simulink model "control_clasic"  (R2025b)
settings: Solver=VariableStepAuto  StartTime=0.0  StopTime=10  RelTol=1e-3
libraries: slpidlib x2
settings Model: Creator=bogdu  LastModifiedBy=Sficaro

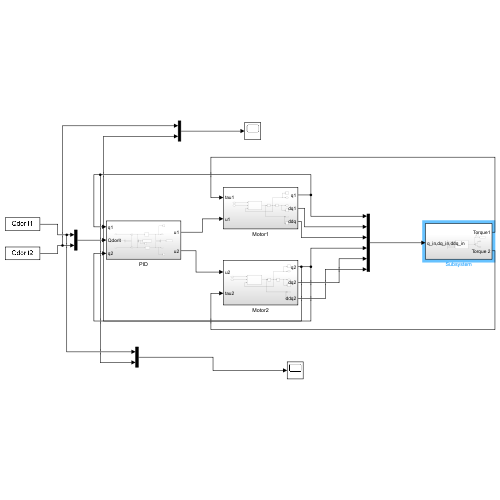
[thumbnail: Simulink's stored preview of the top-level diagram]
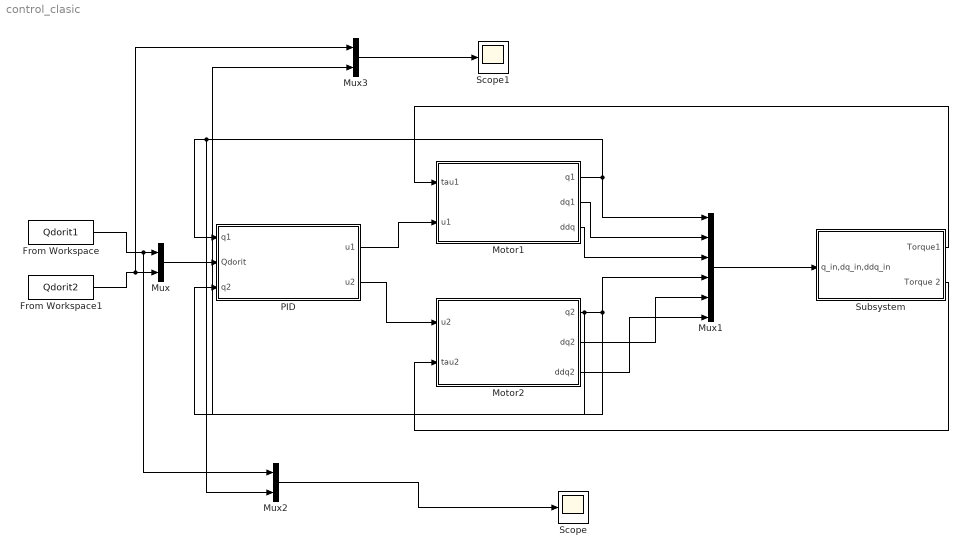
== system control_clasic ==
  From Workspace : FromWorkspace  VariableName=Qdorit1
  From Workspace1 : FromWorkspace  VariableName=Qdorit2
  Motor1 : Subsystem
  Motor2 : Subsystem
  Mux : Mux  Inputs=2
  Mux1 : Mux  Inputs=6
  Mux2 : Mux  Inputs=2
  Mux3 : Mux  Inputs=2
  PID : Subsystem
  Scope : Scope
      settings: ActiveDisplayYMinimum=-1  ActiveDisplayYMaximum=1  DataLoggingVariableName=ScopeData8
  Scope1 : Scope
      settings: ActiveDisplayYMinimum=-0.012500000000000004  ActiveDisplayYMaximum=0.11250000000000007
  Subsystem : Subsystem
  wires:
  From Workspace/1 -> Mux2/1, Mux/1
  From Workspace1/1 -> Mux3/1, Mux/2
  Mux/1 -> PID/2(Qdorit)
  Subsystem/1(Torque1) -> Motor1/1(tau1)
  Subsystem/2(Torque 2) -> Motor2/2(tau2)
  PID/1(u1) -> Motor1/2(u1)
  PID/2(u2) -> Motor2/1(u2)
  Motor1/1(q1) -> Mux1/1, Mux2/2, PID/1(q1)
  Motor2/1(q2) -> Mux3/2, Mux1/4, PID/3(q2)
  Motor1/2(dq1) -> Mux1/2
  Motor1/3(ddq) -> Mux1/3
  Motor2/2(dq2) -> Mux1/5
  Motor2/3(ddq2) -> Mux1/6
  Mux1/1 -> Subsystem/1(q_in,dq_in,ddq_in)
  Mux2/1 -> Scope/1
  Mux3/1 -> Scope1/1

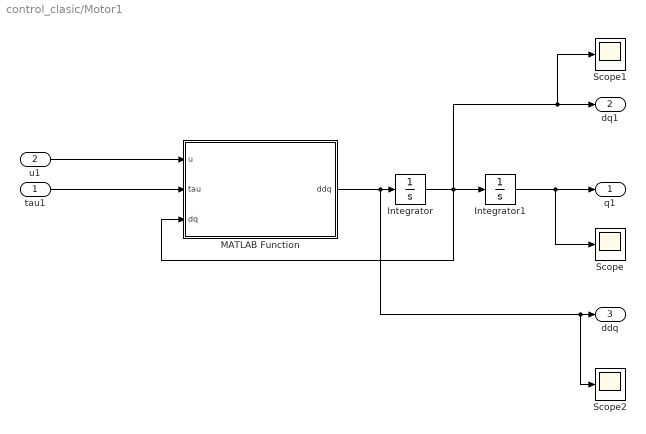
== system control_clasic/Motor1 ==
  tau1 : Inport
  u1 : Inport  Port=2
  Integrator : Integrator
  Integrator1 : Integrator
  MATLAB Function : MATLAB Function  TreatAsAtomicUnit=on
  Scope : Scope
      settings: ActiveDisplayYMinimum=-1  ActiveDisplayYMaximum=1
  Scope1 : Scope
      settings: ActiveDisplayYMinimum=-1  ActiveDisplayYMaximum=1
  Scope2 : Scope
      settings: ActiveDisplayYMinimum=-1  ActiveDisplayYMaximum=1  DataLoggingVariableName=ScopeData2
  q1 : Outport
  dq1 : Outport  Port=2
  ddq : Outport  Port=3
  wires:
  MATLAB Function/1(ddq) -> Scope2/1, ddq/1, Integrator/1
  Integrator1/1 -> Scope/1, q1/1
  Integrator/1 -> Scope1/1, dq1/1, Integrator1/1, MATLAB Function/3(dq)
  u1/1 -> MATLAB Function/1(u)
  tau1/1 -> MATLAB Function/2(tau)

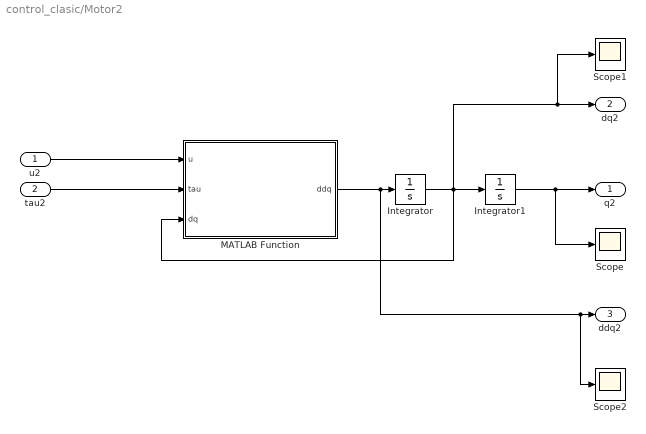
== system control_clasic/Motor2 ==
  u2 : Inport
  tau2 : Inport  Port=2
  Integrator : Integrator
  Integrator1 : Integrator
  MATLAB Function : MATLAB Function  TreatAsAtomicUnit=on
  Scope : Scope
      settings: ActiveDisplayYMinimum=-0.01248  ActiveDisplayYMaximum=0.11232  DataLoggingVariableName=ScopeData3
  Scope1 : Scope
      settings: ActiveDisplayYMinimum=-0.00187  ActiveDisplayYMaximum=0.01686  DataLoggingVariableName=ScopeData4
  Scope2 : Scope
      settings: ActiveDisplayYMinimum=-0.00957  ActiveDisplayYMaximum=0.00897  DataLoggingVariableName=ScopeData5
  q2 : Outport
  dq2 : Outport  Port=2
  ddq2 : Outport  Port=3
  wires:
  Integrator/1 -> Scope1/1, dq2/1, Integrator1/1, MATLAB Function/3(dq)
  tau2/1 -> MATLAB Function/2(tau)
  u2/1 -> MATLAB Function/1(u)
  Integrator1/1 -> Scope/1, q2/1
  MATLAB Function/1(ddq) -> Scope2/1, ddq2/1, Integrator/1

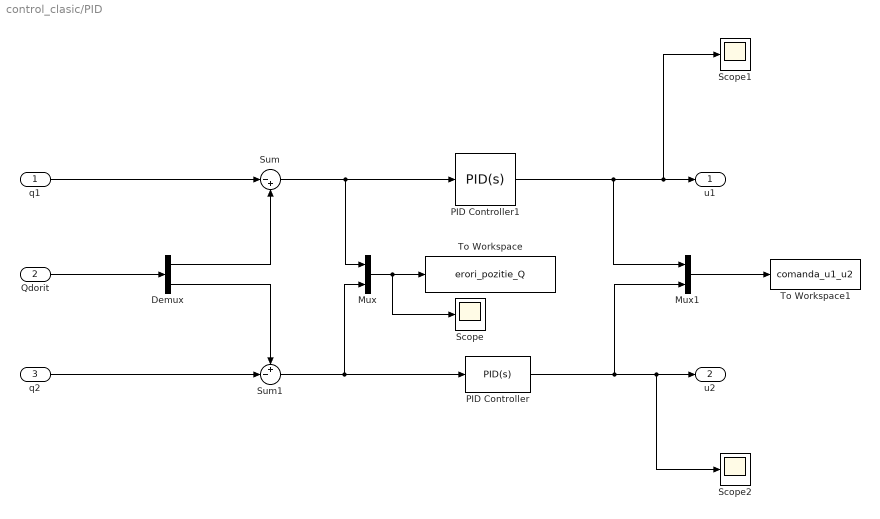
== system control_clasic/PID ==
  q1 : Inport
  Qdorit : Inport  Port=2
  q2 : Inport  Port=3
  Demux : Demux  Outputs=2
  Mux : Mux  Inputs=2
  Mux1 : Mux  Inputs=2
  PID Controller : slpidlib/PID Controller  Controller=PID  Form=Parallel  TimeDomain=Continuous-time  UseExternalTs=off  SampleTime=-1  IntegratorMethod=Forward Euler  FilterMethod=Forward Euler  ControllerParametersSource=internal  P=7000  I=10  UseKiTs=off  D=2  UseExternalDerivativeSource=off  N=250  UseFilter=on  TunerSelectOption=Transfer Function Based (PID Tuner App)  InitialConditionSource=internal  InitialConditionForIntegrator=0  InitialConditionForFilter=0  DifferentiatorICPrevScaledInput=0  ExternalReset=none  TrackingMode=off  Kt=1  LimitOutput=on  SatLimitsSource=internal  UpperSaturationLimit=24  LowerSaturationLimit=-24  LinearizeAsGain=on  AntiWindupMode=none  Kb=1  LimitIntegrator=off  UpperIntegratorSaturationLimit=inf  LowerIntegratorSaturationLimit=-inf  POutMin=[]  POutMax=[]  IOutMin=[]  IOutMax=[]  DOutMin=[]  DOutMax=[]  NOutMin=[]  NOutMax=[]  SumOutMin=[]  SumOutMax=[]  SaturationOutMin=[]  SaturationOutMax=[]  PParamMin=[]  PParamMax=[]  IParamMin=[]  IParamMax=[]  DParamMin=[]  DParamMax=[]  NParamMin=[]  NParamMax=[]  KbParamMin=[]  KbParamMax=[]  KtParamMin=[]  KtParamMax=[]  KbOutMin=[]  KbOutMax=[]  KtOutMin=[]  KtOutMax=[]  IntegratorOutMin=[]  IntegratorOutMax=[]  FilterOutMin=[]  FilterOutMax=[]  SumI1OutMin=[]  SumI1OutMax=[]  SumI2OutMin=[]  SumI2OutMax=[]  SumI3OutMin=[]  SumI3OutMax=[]  SumI4OutMin=[]  SumI4OutMax=[]  SumDOutMin=[]  SumDOutMax=[]  DifferentiatorOutMin=[]  DifferentiatorOutMax=[]  FilterDiffOutCoefMin=[]  FilterDiffOutCoefMax=[]  ReciprocalOutMin=[]  ReciprocalOutMax=[]  SumDenOutMin=[]  SumDenOutMax=[]  SumNumOutMin=[]  SumNumOutMax=[]  DivideOutMin=[]  DivideOutMax=[]  UdiffTsProdOutMin=[]  UdiffTsProdOutMax=[]  NTsProdOutMin=[]  NTsProdOutMax=[]  UintegralTsProdOutMin=[]  UintegralTsProdOutMax=[]  UngainTsProdOutMin=[]  UngainTsProdOutMax=[]  ClampingZeroOutDataTypeStr=Inherit: Inherit via back propagation  ClampingZeroOutMin=[]  ClampingZeroOutMax=[]  FilterDenConstantOutDataTypeStr=Inherit: Inherit via back propagation  FilterDenConstantOutMin=[]  FilterDenConstantOutMax=[]  PCopyOutDataTypeStr=Inherit: Inherit via back propagation  PCopyOutMin=[]  PCopyOutMax=[]  NCopyOutDataTypeStr=Inherit: Inherit via back propagation  NCopyOutMin=[]  NCopyOutMax=[]  IntegratorContinuousStateAttributes=''  IntegratorStateMustResolveToSignalObject=off  IntegratorRTWStateStorageClass=Auto  FilterContinuousStateAttributes=''  FilterStateMustResolveToSignalObject=off  FilterRTWStateStorageClass=Auto  ParallelPVariant=InternalParameters  IdealPVariant=Disabled  IVariant=InternalParameters  DVariant=InternalParameters  IntegratorVariant=Continuous  SatVariant=Enabled  AWVariant=Passthrough  PCopyVariant=Disabled  TRVariant=Disabled  FdbkBlocksVariant=Forward  IdealPFdbkVariant=Disabled  SatFdbkVariant=Disabled  DerivativeFilterVariant=ContFilter  NVariant=InternalParameters  NCopyVariant=Disabled  FilterICVariant=InternalICsFilter  IntegratorICVariant=InternalICs  ExternalResetVariant=Disabled  TRSumVariant=Passthrough  SumFdbkVariant=Disabled  SumVariant=Sum_PID  TsampFilterVariant=InternalTs  TsampNgainVariant=Passthrough  TsampIntegralVariant=Disabled_SignalSpec  ExternalSaturationOutDataTypeStr=Inherit: Same as second input  DerivativeSourceVariant=ErrorSignal  PreIntVariant=InternalPreInt
  PID Controller1 : slpidlib/PID Controller  Controller=PID  Form=Parallel  TimeDomain=Continuous-time  UseExternalTs=off  SampleTime=-1  IntegratorMethod=Forward Euler  FilterMethod=Forward Euler  ControllerParametersSource=internal  P=1000  I=3  UseKiTs=off  D=1  UseExternalDerivativeSource=off  N=100  UseFilter=on  TunerSelectOption=Transfer Function Based (PID Tuner App)  InitialConditionSource=internal  InitialConditionForIntegrator=0  InitialConditionForFilter=0  DifferentiatorICPrevScaledInput=0  ExternalReset=none  TrackingMode=off  Kt=1  LimitOutput=on  SatLimitsSource=internal  UpperSaturationLimit=24  LowerSaturationLimit=-24  LinearizeAsGain=on  AntiWindupMode=none  Kb=1  LimitIntegrator=off  UpperIntegratorSaturationLimit=inf  LowerIntegratorSaturationLimit=-inf  POutMin=[]  POutMax=[]  IOutMin=[]  IOutMax=[]  DOutMin=[]  DOutMax=[]  NOutMin=[]  NOutMax=[]  SumOutMin=[]  SumOutMax=[]  SaturationOutMin=[]  SaturationOutMax=[]  PParamMin=[]  PParamMax=[]  IParamMin=[]  IParamMax=[]  DParamMin=[]  DParamMax=[]  NParamMin=[]  NParamMax=[]  KbParamMin=[]  KbParamMax=[]  KtParamMin=[]  KtParamMax=[]  KbOutMin=[]  KbOutMax=[]  KtOutMin=[]  KtOutMax=[]  IntegratorOutMin=[]  IntegratorOutMax=[]  FilterOutMin=[]  FilterOutMax=[]  SumI1OutMin=[]  SumI1OutMax=[]  SumI2OutMin=[]  SumI2OutMax=[]  SumI3OutMin=[]  SumI3OutMax=[]  SumI4OutMin=[]  SumI4OutMax=[]  SumDOutMin=[]  SumDOutMax=[]  DifferentiatorOutMin=[]  DifferentiatorOutMax=[]  FilterDiffOutCoefMin=[]  FilterDiffOutCoefMax=[]  ReciprocalOutMin=[]  ReciprocalOutMax=[]  SumDenOutMin=[]  SumDenOutMax=[]  SumNumOutMin=[]  SumNumOutMax=[]  DivideOutMin=[]  DivideOutMax=[]  UdiffTsProdOutMin=[]  UdiffTsProdOutMax=[]  NTsProdOutMin=[]  NTsProdOutMax=[]  UintegralTsProdOutMin=[]  UintegralTsProdOutMax=[]  UngainTsProdOutMin=[]  UngainTsProdOutMax=[]  ClampingZeroOutDataTypeStr=Inherit: Inherit via back propagation  ClampingZeroOutMin=[]  ClampingZeroOutMax=[]  FilterDenConstantOutDataTypeStr=Inherit: Inherit via back propagation  FilterDenConstantOutMin=[]  FilterDenConstantOutMax=[]  PCopyOutDataTypeStr=Inherit: Inherit via back propagation  PCopyOutMin=[]  PCopyOutMax=[]  NCopyOutDataTypeStr=Inherit: Inherit via back propagation  NCopyOutMin=[]  NCopyOutMax=[]  IntegratorContinuousStateAttributes=''  IntegratorStateMustResolveToSignalObject=off  IntegratorRTWStateStorageClass=Auto  FilterContinuousStateAttributes=''  FilterStateMustResolveToSignalObject=off  FilterRTWStateStorageClass=Auto  ParallelPVariant=InternalParameters  IdealPVariant=Disabled  IVariant=InternalParameters  DVariant=InternalParameters  IntegratorVariant=Continuous  SatVariant=Enabled  AWVariant=Passthrough  PCopyVariant=Disabled  TRVariant=Disabled  FdbkBlocksVariant=Forward  IdealPFdbkVariant=Disabled  SatFdbkVariant=Disabled  DerivativeFilterVariant=ContFilter  NVariant=InternalParameters  NCopyVariant=Disabled  FilterICVariant=InternalICsFilter  IntegratorICVariant=InternalICs  ExternalResetVariant=Disabled  TRSumVariant=Passthrough  SumFdbkVariant=Disabled  SumVariant=Sum_PID  TsampFilterVariant=InternalTs  TsampNgainVariant=Passthrough  TsampIntegralVariant=Disabled_SignalSpec  ExternalSaturationOutDataTypeStr=Inherit: Same as second input  DerivativeSourceVariant=ErrorSignal  PreIntVariant=InternalPreInt
  Scope : Scope
      settings: ActiveDisplayYMinimum=-0.0018209575593210454  ActiveDisplayYMaximum=0.016388618033889413  DataLoggingVariableName=ScopeData7
  Scope1 : Scope
      settings: ActiveDisplayYMinimum=-1  ActiveDisplayYMaximum=1  DataLoggingVariableName=ScopeData2
  Scope2 : Scope
      settings: ActiveDisplayYMinimum=-1  ActiveDisplayYMaximum=1  DataLoggingVariableName=ScopeData3
  Sum : Sum  Inputs=|-+
  Sum1 : Sum  Inputs=+-|
  To Workspace : ToWorkspace  VariableName=erori_pozitie_Q  SaveFormat=Timeseries  SampleTime=-1
  To Workspace1 : ToWorkspace  VariableName=comanda_u1_u2  SaveFormat=Timeseries  SampleTime=-1
  u1 : Outport
  u2 : Outport  Port=2
  wires:
  Qdorit/1 -> Demux/1
  Demux/1 -> Sum/2
  Demux/2 -> Sum1/1
  Sum1/1 -> PID Controller/1, Mux/2
  Sum/1 -> PID Controller1/1, Mux/1
  Mux/1 -> Scope/1, To Workspace/1
  PID Controller1/1 -> Mux1/1, Scope1/1, u1/1
  PID Controller/1 -> Mux1/2, Scope2/1, u2/1
  Mux1/1 -> To Workspace1/1
  q1/1 -> Sum/1
  q2/1 -> Sum1/2

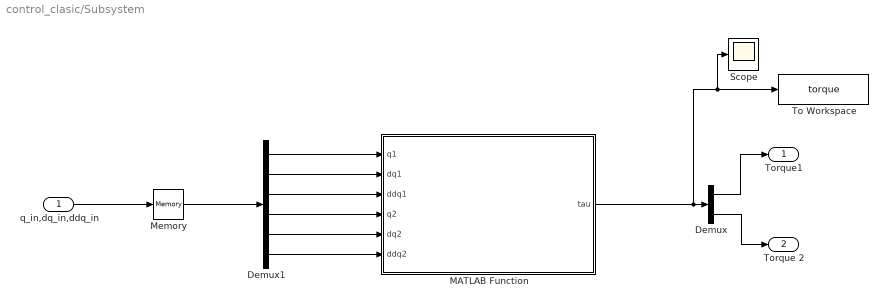
== system control_clasic/Subsystem ==
  q_in,dq_in,ddq_in : Inport
  Demux : Demux  Outputs=2
  Demux1 : Demux  Outputs=6
  MATLAB Function : MATLAB Function  TreatAsAtomicUnit=on
  Memory : Memory
  Scope : Scope
      settings: ActiveDisplayYMinimum=-221.19935628386966  ActiveDisplayYMaximum=198.08517151087329  DataLoggingVariableName=ScopeData6
  To Workspace : ToWorkspace  VariableName=torque  SaveFormat=Timeseries  SampleTime=-1
  Torque1 : Outport
  Torque 2 : Outport  Port=2
  wires:
  q_in,dq_in,ddq_in/1 -> Memory/1
  Memory/1 -> Demux1/1
  MATLAB Function/1(tau) -> Scope/1, To Workspace/1, Demux/1
  Demux/1 -> Torque1/1
  Demux/2 -> Torque 2/1
  Demux1/1 -> MATLAB Function/1(q1)
  Demux1/2 -> MATLAB Function/2(dq1)
  Demux1/3 -> MATLAB Function/3(ddq1)
  Demux1/4 -> MATLAB Function/4(q2)
  Demux1/5 -> MATLAB Function/5(dq2)
  Demux1/6 -> MATLAB Function/6(ddq2)

== matlab function control_clasic/Motor2/MATLAB Function ==
  data: u input; tau input; ddq output; dq input
function ddq = Motor_Linear(u, tau, dq)
    % Parametri motor rotativ (identici cu originalul)
    b = 0.1;              % [Nms/rad]
    k_M = 40.4*10^-3;     % [Nm/A]
    randament = 1;
    i_r = 210;
    R = 0.100;            % [Ω]
    J_a = 20*10^-6;     % [kgm²]
    
    % Parametru de conversie rotație → translație
    r = 0.05;             % [m] - raza roții/scrubului (AJUSTEAZĂ!)
    
    % Conversie translație → rotație
    dq = dq / r;                    % viteza unghiulară [rad/s]
    tau = tau * r;                % cuplu extern [Nm]
    
    % Calculul accelerației unghiulare (ca la original)
    factor1 = (b + k_M^2/R) * dq;
    factor2 = tau / (randament * i_r^2);
    factor3 = k_M / (i_r * R) * u;
    
    ddq = 1/J_a * (factor3 - factor1 - factor2);
    
    % Conversie accelerație unghiulară → liniară
    ddq = ddq * r;                  % [m/s²]
end

== matlab function control_clasic/Motor1/MATLAB Function ==
  data: u input; ddq output; tau input; dq input
function ddq = Motor(u, tau, dq)

    b = 0.1; %[Nms/rad]
    k_M = 13.7*10^-3; %[mNm/A]
    randament = 1; 
    i_r = 81;
    R = 0.102; %[ohm]
    J_a = 43*10^-6; %[gcm^2]


    factor1 = (b + k_M^2/R)*dq;
    factor2 = tau/(randament*i_r^2);
    factor3 = k_M / (i_r * R) * u;
    ddq = 1/J_a * (factor3 - factor1 - factor2);

== matlab function control_clasic/Subsystem/MATLAB Function ==
  data: q1 input; dq1 input; tau output; ddq1 input; q2 input; dq2 input; ddq2 input
function tau = tau_compute(q1,dq1, ddq1, q2, dq2, ddq2)
    
    % parametri structura
    mc1 = 0.5;      
    mc2 = 0.5;      
    l1 = 0.4;
    lc2 = 0.1;
    lc1 = 0.2;
    Izz1 = 0.000625;
    Izz2 = 0.00197;
    Ixx_1 = Izz1;
    Ixx_2 = Izz2;
    g=9.81;
   
    % mass inertia
    M = [mc2*l1^2 + 2*mc2*l1*lc2 + 2*mc2*l1*q2 + mc1*lc1^2 + mc2*lc2^2 + 2*mc2*lc2*q2 + mc2*q2^2 + Ixx_1 + Ixx_2,              0;
                                                  0,                                                                           mc2];
    M = M * [ddq1; ddq2];

     % coriolis
    B_coriolis = [2*mc2*(l1 + lc2 + q2); 
                           0];
    
    % centrifugal
    Cn = [           0,                      0; 
         -mc2*(l1 + lc2 + q2),                0];
    % coriolis + centrifugal
    N = Cn*[dq1^2; dq2^2] + B_coriolis*dq1*dq2;

    G = [g*mc2*(cos(q1)*(l1 + q2) + lc2*cos(q1)) + g*lc1*mc1*cos(q1); 
                               g*mc2*sin(q1)];

    tau = M + N + G;
